simulink model "MainController_Behavior"  (R2025b)
settings: Solver=VariableStepAuto  StartTime=0.0  StopTime=10.0  RelTol=1e-3
settings Model: Creator=prati  LastModifiedBy=prati

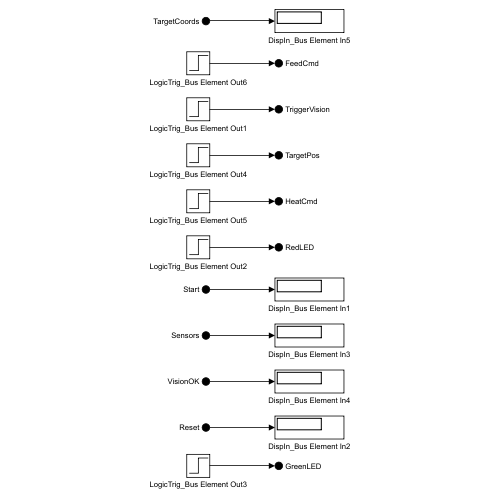
[thumbnail: Simulink's stored preview of the top-level diagram]
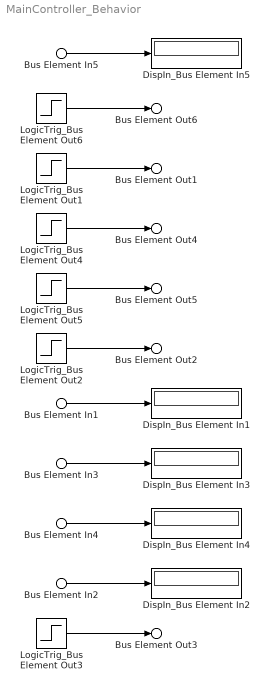
== system MainController_Behavior ==
  Bus Element In1 : Inport  PortName=Start
  Bus Element In2 : Inport  Port=2  PortName=Reset
  Bus Element In3 : Inport  Port=3  PortName=Sensors
  Bus Element In4 : Inport  Port=4  PortName=VisionOK
  Bus Element In5 : Inport  Port=5  PortName=TargetCoords
  DispIn_Bus Element In{1..5} (5 alike) : Display
  LogicTrig_Bus Element Out{1..6} (6 alike) : Step  Time=0  SampleTime=0
  Bus Element Out1 : Outport  PortName=TriggerVision
  Bus Element Out2 : Outport  Port=2  PortName=RedLED
  Bus Element Out3 : Outport  Port=3  PortName=GreenLED
  Bus Element Out4 : Outport  Port=4  PortName=TargetPos
  Bus Element Out5 : Outport  Port=5  PortName=HeatCmd
  Bus Element Out6 : Outport  Port=6  PortName=FeedCmd
  wires:
  Bus Element In2/1 -> DispIn_Bus Element In2/1
  LogicTrig_Bus Element Out1/1 -> Bus Element Out1/1
  Bus Element In5/1 -> DispIn_Bus Element In5/1
  LogicTrig_Bus Element Out5/1 -> Bus Element Out5/1
  LogicTrig_Bus Element Out6/1 -> Bus Element Out6/1
  LogicTrig_Bus Element Out4/1 -> Bus Element Out4/1
  LogicTrig_Bus Element Out2/1 -> Bus Element Out2/1
  Bus Element In3/1 -> DispIn_Bus Element In3/1
  Bus Element In1/1 -> DispIn_Bus Element In1/1
  Bus Element In4/1 -> DispIn_Bus Element In4/1
  LogicTrig_Bus Element Out3/1 -> Bus Element Out3/1
